simulink model "Sim_BPSK_2"  (Simulink 10.1)
settings: Solver=VariableStepAuto  StartTime=0.0  StopTime=50  RelTol=1e-3
libraries: commdigbbndpm3 x2, commchan3 x1, commrandsrc2 x1
settings Model: Creator=mawenjian  LastModifiedBy=mawenjian
settings DataIOCC: SaveFormat=Dataset  ReturnWorkspaceOutputs=on
settings OptimizationCC: LifeSpan=auto
settings DebuggingCC: UnderspecifiedInitializationDetection=Simplified  MergeDetectMultiDrivingBlocksExec=error  SFUnexpectedBacktrackingDiag=error  SFNoUnconditionalDefaultTransitionDiag=error  SFExecutionAtInitializationDiag=warning  ArithmeticOperatorsInVariantConditions=error
settings HardwareCC: ProdBitPerPointer=64  ProdBitPerSizeT=64  ProdBitPerPtrDiffT=64  ProdLargestAtomicFloat=Float  ProdIntDivRoundTo=Zero  ProdEndianess=LittleEndian  ProdWordSize=64  ProdHWDeviceType=Intel->x86-64 (Windows64)
settings ModelReferenceCC: PropagateSignalLabelsOutOfModel=on
settings SFSimCC: SimUseLocalCustomCode=on  CustomCodeUndefinedFunction=FilterOut
settings RTWCC: RTWUseLocalCustomCode=on
settings CodeAppCC: StateflowObjectComments=off
settings GRTTargetCC: TargetLangStandard=C99 (ISO)  CombineOutputUpdateFcns=on  GRTInterface=off
settings ConfigComp: CovMetricSettings=dwe  CovHtmlReporting=off  CovSaveCumulativeToWorkspaceVar=off  CovSaveSingleToWorkspaceVar=off  CovExternalEMLEnable=on

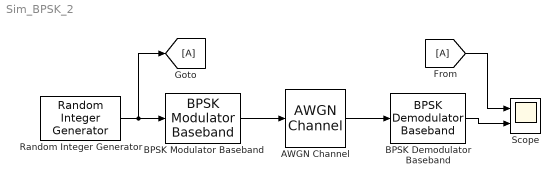
== system Sim_BPSK_2 ==
  AWGN Channel : commchan3/AWGN Channel  InputProcessing=Columns as channels (frame based)  seed=67  noiseMode="Signal to noise ratio  (Eb/No)"  EbNodB=-10  EsNodB=4  SNRdB=10  bitsPerSym=1  Ps=1  Tsym=1  variance=1
  BPSK Demodulator Baseband : commdigbbndpm3/BPSK Demodulator Baseband  DecType=Hard decision  VarSource=Dialog  Variance=1  Ph=0  outDtype=Inherit via internal rule  derotateFactorWordLen=16  derotateFactorDataTypeStr=Inherit: Same word length as input  derotateFactorLastDataTypeStr=Inherit: Same word length as input
  BPSK Modulator Baseband : commdigbbndpm3/BPSK Modulator Baseband  Ph=0  outDtype=double  outWordLen=16  outUDDataType=sfix(16)  outFracLenMode=Best precision  outFracLen=15  outDataTypeStr=double  outLastDataTypeStr=double
  Random Integer Generator : commrandsrc2/Random Integer Generator  mul=2  seed=37  Ts=1  frameBased=off  sampPerFrame=1000  orient=off  outDataType=boolean
      settings: SourceProductBaseCode=CM
  Scope : Scope  NumInputPorts=2
  wires:
  Random Integer Generator/1 -> [A], BPSK Modulator Baseband/1
  BPSK Modulator Baseband/1 -> AWGN Channel/1
  AWGN Channel/1 -> BPSK Demodulator Baseband/1
  BPSK Demodulator Baseband/1 -> Scope/2
  [A] -> Scope/1
